simulink model "power_system"  (R2026b)
settings: Solver=VariableStepAuto  StopTime=param.sim.simlength
model workspace (MAT data in the model file):
  phi = 0.785398163397
values from neighbouring files (symbols this model uses):
  param = struct()    [init_model.m]
undefined symbols (not defined in the file or in its folder): dmavg_flt, simple_moving_average_filter
libraries: fl_lib x37, nesl_utility x22, single_phase_transformer_lib x3, saturable_single_phase_transformer x3, power_meter_iec x2, three_phase_transformer_lib x2, eeGeneralControl x2, moving_average_filter x1, moving_average_filter_cc x1, simulink x1, three_phase_voltage_with_frt_emulator x1, three_phase_rl_load x1
(part 1 of 2)
settings Model: Creator=dbagn  LastModifiedBy=d.bagnara
settings SFSimCC: SimCustomHeaderCode=|
  | #include "rpi.h"
  | #include "mavgflt.h"
  | #include "mavgflt_simulink.h"
  | #include "mavgflts.h"
  | #include "mavgflts_simulink.h"
  | #include "dsmavgflt.h"
  | #include "dsmavgflt_simulink.h"
  | #include "bemf_obsv.h"
  | #include "bemf_obsv_simulink.h"
  | #include "bemf_obsv_load_est.h"
  | #include "bemf_obsv_load_est_simulink.h"
  | #include "dqvector_pi.h"
  | #include "dqvector_pi_simulink.h"
  | #include "sv_pwm_simulink.h"
  | #include "sv_pwm.h"
  | #include "first_harmonic_tracker.h"
  | #include "first_harmonic_tracker_simulink.h"
  | #include "dqpll_thyr.h"
  | #include "dqpll_thyr_simulink.h"
  | #include "dqpll_grid.h"
  | #include "dqpll_grid_simulink.h"
  | #include "linear_double_integrator_observer_simulink.h"
  | #include "linear_double_integrator_observer.h"
settings SFSimCC: SimUserIncludeDirs=|
  | include
  | src
settings SFSimCC: SimUserSources=|
  | "rpi.c"
  | "mavgflt_simulink.c"
  | "mavgflt.c"
  | "mavgflts_simulink.c"
  | "mavgflts.c"
  | "dsmavgflt_simulink.c"
  | "dsmavgflt.c"
  | "bemf_obsv_simulink.c"
  | "bemf_obsv.c"
  | "bemf_obsv_load_est_simulink.c"
  | "bemf_obsv_load_est.c"
  | "dqvector_pi.c"
  | "dqvector_pi_simulink.c"
  | "sv_pwm_simulink.c"
  | "sv_pwm.c"
  | "first_harmonic_tracker_simulink.c"
  | "first_harmonic_tracker.c"
  | "dqpll_thyr_simulink.c"
  | "dqpll_thyr.c"
  | "dqpll_grid_simulink.c"
  | "dqpll_grid.c"
  | "linear_double_integrator_observer_simulink.c"
  | "linear_double_integrator_observer.c"
settings SimscapeCC: SimscapeUseEnergyAccounting=off

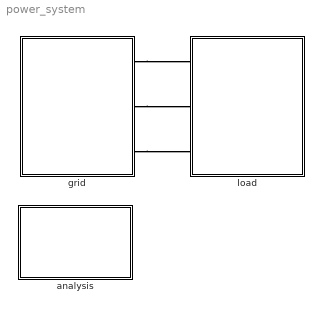
== system power_system ==
  analysis : Subsystem
  grid : Subsystem
  load : Subsystem
  connections:
  grid/RConn1 -- load/LConn1
  grid/RConn2 -- load/LConn2
  grid/RConn3 -- load/LConn3

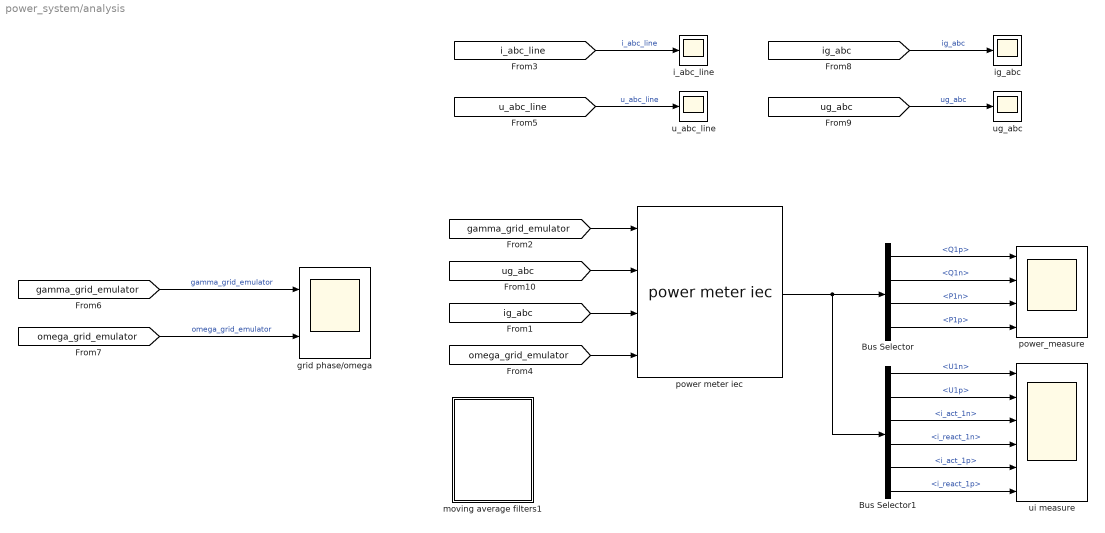
== system power_system/analysis ==
  Bus Selector : BusSelector  OutputSignals=Q1p,Q1n,P1n,P1p
  Bus Selector1 : BusSelector  OutputSignals=U1n,U1p,i_act_1n,i_react_1n,i_act_1p,i_react_1p
  grid phase/omega : Scope  NumInputPorts=2
      settings: ActiveDisplayYMinimum=-3.926953707550084  ActiveDisplayYMaximum=3.9269067422486352  DataLoggingVariableName=ScopeData3
  i_abc_line : Scope
      settings: ActiveDisplayYMinimum=-68.948090283299308  ActiveDisplayYMaximum=59.727285723031869  DataLoggingVariableName=ScopeData4
  ig_abc : Scope
      settings: ActiveDisplayYMinimum=-1  ActiveDisplayYMaximum=1  DataLoggingVariableName=ScopeData6
  moving average filters1 : Subsystem
  power meter iec : power_meter_iec/power meter iec  period=10/param.grid.emu.fgrid_nom  ts=param.glb_time.tc  enable_time=0.025
  power_measure : Scope  NumInputPorts=4
      settings: ActiveDisplayYMinimum=-20130.529238289768  ActiveDisplayYMaximum=181174.76314460795
  u_abc_line : Scope
      settings: ActiveDisplayYMinimum=-704.22830105013838  ActiveDisplayYMaximum=704.22830105010917  DataLoggingVariableName=ScopeData5
  ug_abc : Scope
      settings: ActiveDisplayYMinimum=-698.03378054285679  ActiveDisplayYMaximum=698.02521447934464  DataLoggingVariableName=ScopeData7
  ui measure : Scope  NumInputPorts=6
      settings: ActiveDisplayString=6  ActiveDisplayYMinimum=48.674141527663735  ActiveDisplayYMaximum=144.89470062623792
  wires:
  Bus Selector1/5 -> ui measure/5  "<i_act_1p>"
  Bus Selector/2 -> power_measure/2  "<Q1n>"
  [u_abc_line] -> u_abc_line/1  "u_abc_line"
  [i_abc_line] -> i_abc_line/1  "i_abc_line"
  [ig_abc] -> ig_abc/1  "ig_abc"
  [ug_abc] -> ug_abc/1  "ug_abc"
  Bus Selector1/3 -> ui measure/3  "<i_act_1n>"
  Bus Selector/1 -> power_measure/1  "<Q1p>"
  Bus Selector1/6 -> ui measure/6  "<i_react_1p>"
  Bus Selector1/4 -> ui measure/4  "<i_react_1n>"
  [ug_abc] -> power meter iec/2
  Bus Selector/3 -> power_measure/3  "<P1n>"
  [omega_grid_emulator] -> power meter iec/4
  [ig_abc] -> power meter iec/3
  [gamma_grid_emulator] -> power meter iec/1
  Bus Selector1/1 -> ui measure/1  "<U1n>"
  Bus Selector/4 -> power_measure/4  "<P1p>"
  [omega_grid_emulator] -> grid phase/omega/2  "omega_grid_emulator"
  [gamma_grid_emulator] -> grid phase/omega/1  "gamma_grid_emulator"
  power meter iec/1 -> Bus Selector/1, Bus Selector1/1
  Bus Selector1/2 -> ui measure/2  "<U1p>"

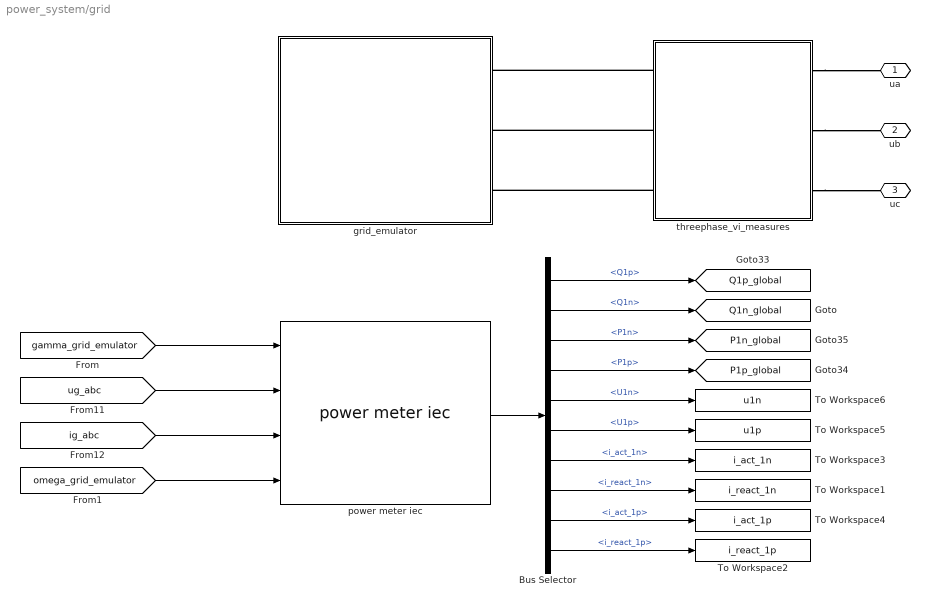
== system power_system/grid ==
  Bus Selector : BusSelector  OutputSignals=Q1p,Q1n,P1n,P1p,U1n,U1p,i_act_1n,i_react_1n,i_act_1p,i_react_1p
  To Workspace1 : ToWorkspace  VariableName=i_react_1n  SampleTime=param.glb_time.ts_afe
      settings: MaxDataPoints=param.glb_time.Ns_afe
  To Workspace2 : ToWorkspace  VariableName=i_react_1p  SampleTime=param.glb_time.ts_afe
      settings: MaxDataPoints=param.glb_time.Ns_afe
  To Workspace3 : ToWorkspace  VariableName=i_act_1n  SampleTime=param.glb_time.ts_afe
      settings: MaxDataPoints=param.glb_time.Ns_afe
  To Workspace4 : ToWorkspace  VariableName=i_act_1p  SampleTime=param.glb_time.ts_afe
      settings: MaxDataPoints=param.glb_time.Ns_afe
  To Workspace5 : ToWorkspace  VariableName=u1p  SampleTime=param.glb_time.ts_afe
      settings: MaxDataPoints=param.glb_time.Ns_afe
  To Workspace6 : ToWorkspace  VariableName=u1n  SampleTime=param.glb_time.ts_afe
      settings: MaxDataPoints=param.glb_time.Ns_afe
  grid_emulator : Subsystem
  power meter iec : power_meter_iec/power meter iec  period=pi/param.grid.emu.omega_grid_nom  ts=param.glb_time.tc  enable_time=0.025
  threephase_vi_measures : Subsystem
  ua : PMIOPort  Side=Right
  ub : PMIOPort  Port=2  Side=Right
  uc : PMIOPort  Port=3  Side=Right
  tag scope: P1n_global=global, P1p_global=global, Q1n_global=global, Q1p_global=global
  wires:
  power meter iec/1 -> Bus Selector/1
  Bus Selector/1 -> [Q1p_global]  "<Q1p>"
  Bus Selector/2 -> [Q1n_global]  "<Q1n>"
  Bus Selector/3 -> [P1n_global]  "<P1n>"
  Bus Selector/4 -> [P1p_global]  "<P1p>"
  Bus Selector/5 -> To Workspace6/1  "<U1n>"
  Bus Selector/6 -> To Workspace5/1  "<U1p>"
  Bus Selector/7 -> To Workspace3/1  "<i_act_1n>"
  Bus Selector/8 -> To Workspace1/1  "<i_react_1n>"
  Bus Selector/9 -> To Workspace4/1  "<i_act_1p>"
  Bus Selector/10 -> To Workspace2/1  "<i_react_1p>"
  [gamma_grid_emulator] -> power meter iec/1
  [ug_abc] -> power meter iec/2
  [ig_abc] -> power meter iec/3
  [omega_grid_emulator] -> power meter iec/4
  connections:
  threephase_vi_measures/LConn3 -- grid_emulator/RConn3
  threephase_vi_measures/LConn1 -- grid_emulator/RConn1
  threephase_vi_measures/RConn2 -- ub/RConn1
  threephase_vi_measures/LConn2 -- grid_emulator/RConn2
  threephase_vi_measures/RConn1 -- ua/RConn1
  threephase_vi_measures/RConn3 -- uc/RConn1

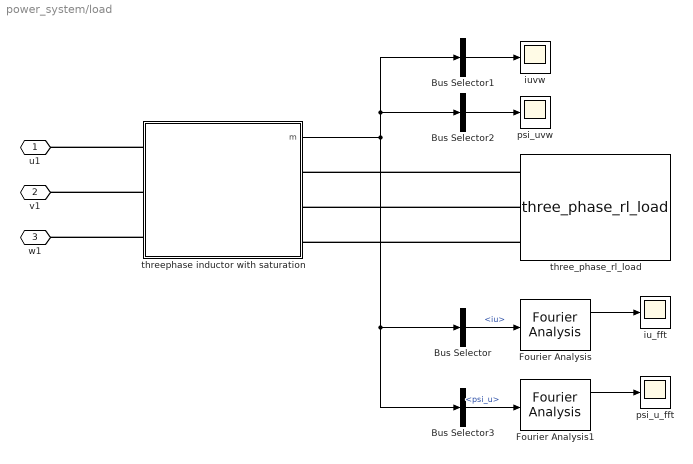
== system power_system/load ==
  Bus Selector : BusSelector  OutputSignals=iu
  Bus Selector1 : BusSelector  OutputSignals=iu,iv,iw  OutputAsBus=on
  Bus Selector2 : BusSelector  OutputSignals=psi_u,psi_v,psi_w  OutputAsBus=on
  Bus Selector3 : BusSelector  OutputSignals=psi_u
  Fourier Analysis : eeGeneralControl/Fourier Analysis  f=50  n=[3, 5, 7, 11]  M0=1  Ph0=0  BufferSize=8192  Ts=param.glb_time.ts_afe
      settings: LibrarySourceBlock=ee_sl_lib/General Control/Fourier Analysis
  Fourier Analysis1 : eeGeneralControl/Fourier Analysis  f=50  n=[3, 5, 7, 11]  M0=1  Ph0=0  BufferSize=8192  Ts=param.glb_time.ts_afe
      settings: LibrarySourceBlock=ee_sl_lib/General Control/Fourier Analysis
  iu_fft : Scope
      settings: ActiveDisplayYMinimum=-45.991562692326895  ActiveDisplayYMaximum=413.93793972331429  DataLoggingVariableName=ScopeData9
  iuvw : Scope
      settings: ActiveDisplayYMinimum=-661.72456988619081  ActiveDisplayYMaximum=615.81940216615919  DataLoggingVariableName=ScopeData8
  psi_u_fft : Scope
      settings: ActiveDisplayYMinimum=-0.2430744341634945  ActiveDisplayYMaximum=0.35456280363081638  DataLoggingVariableName=ScopeData11
  psi_uvw : Scope
      settings: ActiveDisplayYMinimum=-0.33417090779252678  ActiveDisplayYMaximum=0.310988798093905  DataLoggingVariableName=ScopeData10
  three_phase_rl_load : three_phase_rl_load/three_phase_rl_load  Ls1_load_m=param.load.Ls_load(1)  Rs1_load_m=param.load.Rs_load(1)  Ls2_load_m=param.load.Ls_load(2)  Rs2_load_m=param.load.Rs_load(2)  Ls3_load_m=param.load.Ls_load(3)  Rs3_load_m=param.load.Rs_load(3)
  threephase inductor with saturation : Subsystem  mask{LFu_m=param.load.ind.LFu, Rs_m=param.load.ind.Rs, LFu0_m=param.load.ind.LFu0, Rs0_m=param.load.ind.Rs0, isat_m=param.load.ind.isat}
      mask prompts: LFu_m "Positive Sequence Inductance [H]"; Rs_m "Positive Sequence Resistance [Ohm]"; LFu0_m "Zero Sequence Inductance [H]"; Rs0_m "Zero Sequence Resistance [Ohm]"; isat_m "Saturation Current [Arms]"
      mask Display:
      | disp('3P~ind with sat');
      | 
      | port_label('output', 1, 'm');
      | 
      | port_label('lconn', 1, 'u1');
      | port_label('lconn', 2, 'v1');
      | port_label('lconn', 3, 'w1');
      | port_label('rconn', 1, 'u2');
      | port_label('rconn', 2, 'v2');
      | port_label('rconn', 3, 'w2');
  u1 : PMIOPort  Side=Left
  v1 : PMIOPort  Port=2  Side=Left
  w1 : PMIOPort  Port=3  Side=Left
  wires:
  Bus Selector/1 -> Fourier Analysis/1  "<iu>"
  Fourier Analysis/1 -> iu_fft/1
  Bus Selector1/1 -> iuvw/1
  Bus Selector2/1 -> psi_uvw/1
  threephase inductor with saturation/1(m) -> Bus Selector2/1, Bus Selector1/1, Bus Selector3/1, Bus Selector/1
  Fourier Analysis1/1 -> psi_u_fft/1
  Bus Selector3/1 -> Fourier Analysis1/1  "<psi_u>"
  connections:
  threephase inductor with saturation/LConn1 -- u1/RConn1
  threephase inductor with saturation/LConn2 -- v1/RConn1
  threephase inductor with saturation/LConn3 -- w1/RConn1
  three_phase_rl_load/LConn1 -- threephase inductor with saturation/RConn1
  three_phase_rl_load/LConn2 -- threephase inductor with saturation/RConn2
  three_phase_rl_load/LConn3 -- threephase inductor with saturation/RConn3

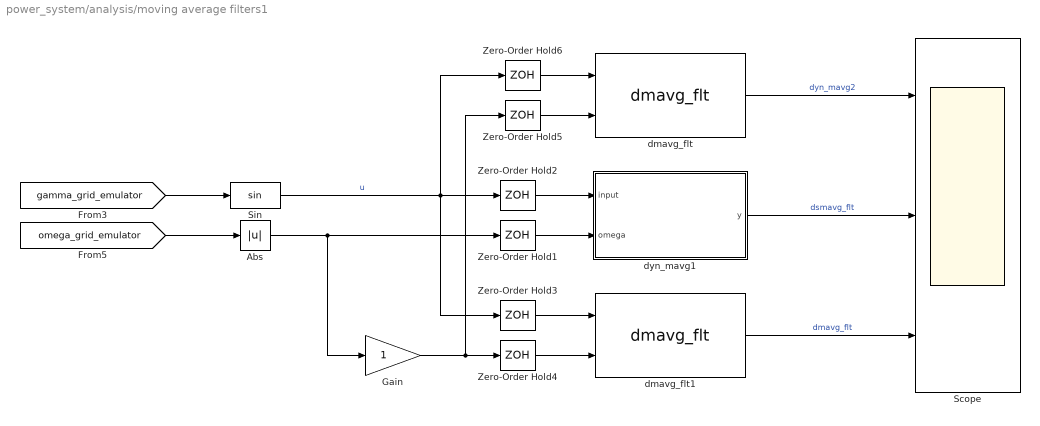
== system power_system/analysis/moving average filters1 ==
  Abs : Abs  SaturateOnIntegerOverflow=off
  Gain : Gain
  Scope : Scope  NumInputPorts=3
      settings: ActiveDisplayYMinimum=-1.2499809265136719  ActiveDisplayYMaximum=1.2499809265136719  DataLoggingVariableName=ScopeData2
  Sin : Trigonometry
  Zero-Order Hold{1..6} (6 alike) : ZeroOrderHold  SampleTime=param.glb_time.ts_afe
  dmavg_flt : moving_average_filter/dmavg_flt  ts=param.glb_time.ts_afe  enable_time=0.025
  dmavg_flt1 : moving_average_filter_cc/dmavg_flt  instance=0  ts=param.glb_time.ts_afe  enable_time=0.025
  dyn_mavg1 : Subsystem  AncestorBlock=simple_moving_average_filter/dmavg_flt  mask{ts=param.glb_time.ts_afe}
      mask prompts: ts "sampling time (s)"
      mask Display:
      | disp('dyn_mavg_flt');
      | port_label('input', 1, 'input');
      | port_label('input', 2, 'omega');
      | port_label('output', 1, 'output');
  wires:
  dyn_mavg1/1(y) -> Scope/2  "dsmavg_flt"
  Zero-Order Hold3/1 -> dmavg_flt1/1
  [gamma_grid_emulator] -> Sin/1
  Zero-Order Hold1/1 -> dyn_mavg1/2(omega)
  Zero-Order Hold4/1 -> dmavg_flt1/2
  dmavg_flt1/1 -> Scope/3  "dmavg_flt"
  [omega_grid_emulator] -> Abs/1
  Zero-Order Hold2/1 -> dyn_mavg1/1(input)
  Sin/1 -> Zero-Order Hold6/1, Zero-Order Hold3/1, Zero-Order Hold2/1  "u"
  Abs/1 -> Zero-Order Hold1/1, Gain/1
  Gain/1 -> Zero-Order Hold5/1, Zero-Order Hold4/1
  Zero-Order Hold6/1 -> dmavg_flt/1
  Zero-Order Hold5/1 -> dmavg_flt/2
  dmavg_flt/1 -> Scope/1  "dyn_mavg2"

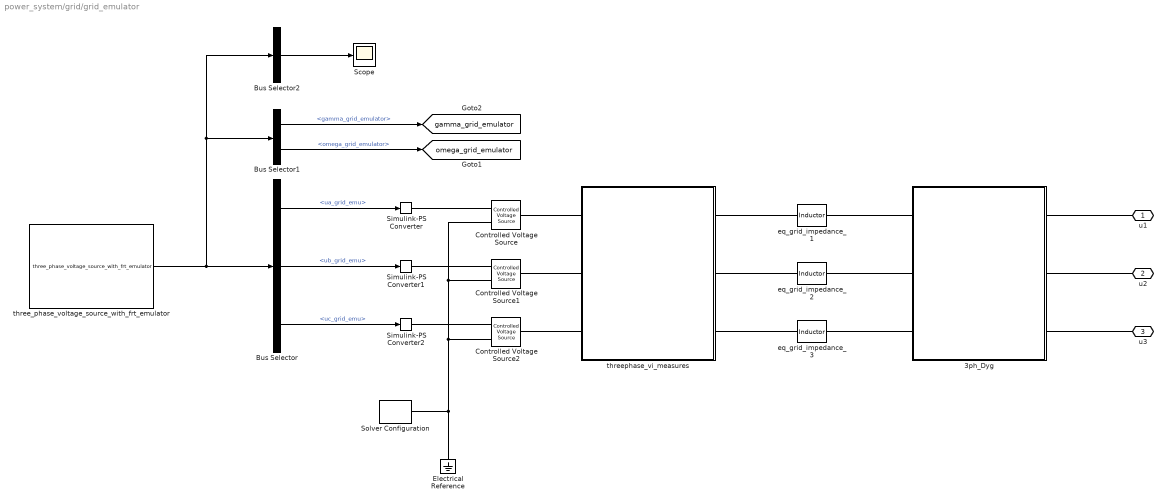
== system power_system/grid/grid_emulator ==
  3ph_Dyg : Subsystem
  Bus Selector : BusSelector  OutputSignals=ua_grid_emu,ub_grid_emu,uc_grid_emu
  Bus Selector1 : BusSelector  OutputSignals=gamma_grid_emulator,omega_grid_emulator
  Bus Selector2 : BusSelector  OutputSignals=vp_xi,vp_eta,vn_xi,vn_eta  OutputAsBus=on
  Controlled Voltage Source : fl_lib/Electrical/Electrical Sources/Controlled Voltage Source
  Controlled Voltage Source1 : fl_lib/Electrical/Electrical Sources/Controlled Voltage Source
  Controlled Voltage Source2 : fl_lib/Electrical/Electrical Sources/Controlled Voltage Source
  Electrical Reference : fl_lib/Electrical/Electrical Elements/Electrical Reference
  Scope : Scope
      settings: ActiveDisplayYMinimum=-323.94501848294675  ActiveDisplayYMaximum=661.97460298693193  DataLoggingVariableName=ScopeData12
  Simulink-PS Converter : nesl_utility/Simulink-PS Converter  PhysicalDomain=network_engine_domain  SubClassName=ps_input  LeftPortType=input  RightPortType=output  PseudoPeriodic=off  Frequencies=[]  NoiseDistribution=none  NoiseParameters=[]  Unit=V  AffineConversion=on  FilteringAndDerivatives=provide  SimscapeFilterOrder=1  InputFilterTimeConstant=0.001  UdotUserProvided=0
  Simulink-PS Converter1 : nesl_utility/Simulink-PS Converter  PhysicalDomain=network_engine_domain  SubClassName=ps_input  LeftPortType=input  RightPortType=output  PseudoPeriodic=off  Frequencies=[]  NoiseDistribution=none  NoiseParameters=[]  Unit=V  AffineConversion=on  FilteringAndDerivatives=provide  SimscapeFilterOrder=1  InputFilterTimeConstant=0.001  UdotUserProvided=0
  Simulink-PS Converter2 : nesl_utility/Simulink-PS Converter  PhysicalDomain=network_engine_domain  SubClassName=ps_input  LeftPortType=input  RightPortType=output  PseudoPeriodic=off  Frequencies=[]  NoiseDistribution=none  NoiseParameters=[]  Unit=V  AffineConversion=on  FilteringAndDerivatives=provide  SimscapeFilterOrder=1  InputFilterTimeConstant=0.001  UdotUserProvided=0
  Solver Configuration : nesl_utility/Solver Configuration  PhysicalDomain=network_engine_domain  SubClassName=solver  LeftPortType=input  RightPortType=generic  Tones=[]  Harmonics=[]  SimulateNoise=off  Profile=off  UseLocalSampling=off  EnableSwitchedLinearOptims=on  FrequencyDomain=off  UseCCode=off  RelTol=0.001  AbsTol=0.001  MinStep=1e-09  ToWorkspace=off  RevertToSquareIcSolve=off  NumHomotopyIterations=100  PhasorMode=off  PhasorModeNumHarmonics=1  ConsistencySolver=NEWTON_FTOL  CanonicalOrdering=UNORDERED  OptimizeIntermediates=UNOPTIMIZED  MulticoreSolverChoice=BACKWARD_EULER  IndexReductionMethod=DerivativeReplacement  DoDC=on  ResidualTolerance=1e-3  ConsistencyTolSource=GLOBAL  ConsistencyAbsTol=0.001  ConsistencyRelTol=0.001  ConsistencyTolFactor=0.001  UseLocalSolver=on  LocalSolverChoice=NE_BACKWARD_EULER_ADVANCER  ResolveIndetEquations=on  FunctionEvalNumThread=1  LocalSolverSampleTime=param.glb_time.tc  DoFixedCost=on  MaxNonlinIter=param.sim.nonlinear_iterations  MaxModeIter=2  ComputeImpulses=off  ImpulseIterations=2  LinearAlgebra=auto  LinearAlgebraNumThread=0  EquationFormulation=NE_TIME_EF  DelaysMemoryBudget=1024  AutomaticFiltering=on  FilteringTimeConstant=0.001  PartitionStorageMethod=AS_NEEDED  PartitionMemoryBudget=1024  PartitionMethod=BALANCED  MultibodyUseLocalSolver=off  MultibodyLocalSolverChoice=ODE1  MultibodyLocalSolverSampleTime=0.001
  eq_grid_impedance_1 : fl_lib/Electrical/Electrical Elements/Inductor  l=param.grid.emu.eq_grid_inductance H  r=param.grid.emu.eq_grid_resistance Ohm  g=1e-9 1/Ohm  i_specify=off  i_priority=None  i=0 A  i_nominal_specify=off  i_nominal_value=1  i_nominal_unit=A  v_specify=off  v_priority=None  v=0 V  v_nominal_specify=off  v_nominal_value=1  v_nominal_unit=V  i_L_specify=off  i_L_priority=High  i_L=0 A  i_L_nominal_specify=off  i_L_nominal_value=1  i_L_nominal_unit=A
  eq_grid_impedance_2 : fl_lib/Electrical/Electrical Elements/Inductor  l=param.grid.emu.eq_grid_inductance H  r=param.grid.emu.eq_grid_resistance Ohm  g=1e-9 1/Ohm  i_specify=off  i_priority=None  i=0 A  i_nominal_specify=off  i_nominal_value=1  i_nominal_unit=A  v_specify=off  v_priority=None  v=0 V  v_nominal_specify=off  v_nominal_value=1  v_nominal_unit=V  i_L_specify=off  i_L_priority=High  i_L=0 A  i_L_nominal_specify=off  i_L_nominal_value=1  i_L_nominal_unit=A
  eq_grid_impedance_3 : fl_lib/Electrical/Electrical Elements/Inductor  l=param.grid.emu.eq_grid_inductance H  r=param.grid.emu.eq_grid_resistance Ohm  g=1e-9 1/Ohm  i_specify=off  i_priority=None  i=0 A  i_nominal_specify=off  i_nominal_value=1  i_nominal_unit=A  v_specify=off  v_priority=None  v=0 V  v_nominal_specify=off  v_nominal_value=1  v_nominal_unit=V  i_L_specify=off  i_L_priority=High  i_L=0 A  i_L_nominal_specify=off  i_L_nominal_value=1  i_L_nominal_unit=A
  three_phase_voltage_source_with_frt_emulator : three_phase_voltage_with_frt_emulator/three_phase_voltage_source_with_frt_emulator  nominal_frequency_m=param.grid.emu.fgrid_nom  nominal_voltage_m=param.grid.emu.us_primary_nom  Vemu_ref_norm_m=param.grid.emu.Vemu_ref_norm  vp_xi_pu_m=param.grid.emu.up_xi_pu_ref  vp_eta_pu_m=param.grid.emu.up_eta_pu_ref  vn_xi_pu_m=param.grid.emu.un_xi_pu_ref  vn_eta_pu_m=param.grid.emu.un_eta_pu_ref  Am=param.grid.emu.sof_50Hz.ss_c.A  Bm=param.grid.emu.sof_50Hz.ss_c.B  Cm=param.grid.emu.sof_50Hz.ss_c.C  enable_frt_1_m=param.grid.frt.enable_frt_1  enable_frt_2_m=param.grid.frt.enable_frt_2  start_time_LVRT_m=param.grid.frt.start_time_LVRT  end_time_LVRT_m=param.grid.frt.end_time_LVRT  deepPOSxi_m=param.grid.frt.deepPOSxi  deepPOSeta_m=param.grid.frt.deepPOSeta  deepNEGxi_m=param.grid.frt.deepNEGxi  deepNEGeta_m=param.grid.frt.deepNEGeta  Amplitude_U_m=param.grid.frt.Amplitude_U  Amplitude_V_m=param.grid.frt.Amplitude_V  Amplitude_W_m=param.grid.frt.Amplitude_W  t_ramp_m=param.grid.frt.t_ramp  Phase_shift_m=param.grid.frt.Phase_shift
  threephase_vi_measures : Subsystem
  u1 : PMIOPort  Side=Right
  u2 : PMIOPort  Port=2  Side=Right
  u3 : PMIOPort  Port=3  Side=Right
  tag scope: gamma_grid_emulator=global, omega_grid_emulator=global
  wires:
  Bus Selector1/2 -> [omega_grid_emulator]  "<omega_grid_emulator>"
  Bus Selector1/1 -> [gamma_grid_emulator]  "<gamma_grid_emulator>"
  Bus Selector/2 -> Simulink-PS Converter1/1  "<ub_grid_emu>"
  Bus Selector/3 -> Simulink-PS Converter2/1  "<uc_grid_emu>"
  three_phase_voltage_source_with_frt_emulator/1 -> Bus Selector1/1, Bus Selector2/1, Bus Selector/1
  Bus Selector/1 -> Simulink-PS Converter/1  "<ua_grid_emu>"
  Bus Selector2/1 -> Scope/1
  connections:
  Simulink-PS Converter/RConn1 -- Controlled Voltage Source/RConn1
  Simulink-PS Converter1/RConn1 -- Controlled Voltage Source1/RConn1
  Simulink-PS Converter2/RConn1 -- Controlled Voltage Source2/RConn1
  Controlled Voltage Source/RConn2 -- Controlled Voltage Source1/RConn2 -- Controlled Voltage Source2/RConn2 -- Electrical Reference/LConn1 -- Solver Configuration/RConn1
  3ph_Dyg/RConn1 -- u1/RConn1
  3ph_Dyg/RConn2 -- u2/RConn1
  3ph_Dyg/RConn3 -- u3/RConn1
  eq_grid_impedance_1/LConn1 -- threephase_vi_measures/RConn1
  eq_grid_impedance_2/LConn1 -- threephase_vi_measures/RConn2
  eq_grid_impedance_3/LConn1 -- threephase_vi_measures/RConn3
  Controlled Voltage Source/LConn1 -- threephase_vi_measures/LConn1
  Controlled Voltage Source1/LConn1 -- threephase_vi_measures/LConn2
  Controlled Voltage Source2/LConn1 -- threephase_vi_measures/LConn3
  3ph_Dyg/LConn1 -- eq_grid_impedance_1/RConn1
  3ph_Dyg/LConn2 -- eq_grid_impedance_2/RConn1
  3ph_Dyg/LConn3 -- eq_grid_impedance_3/RConn1

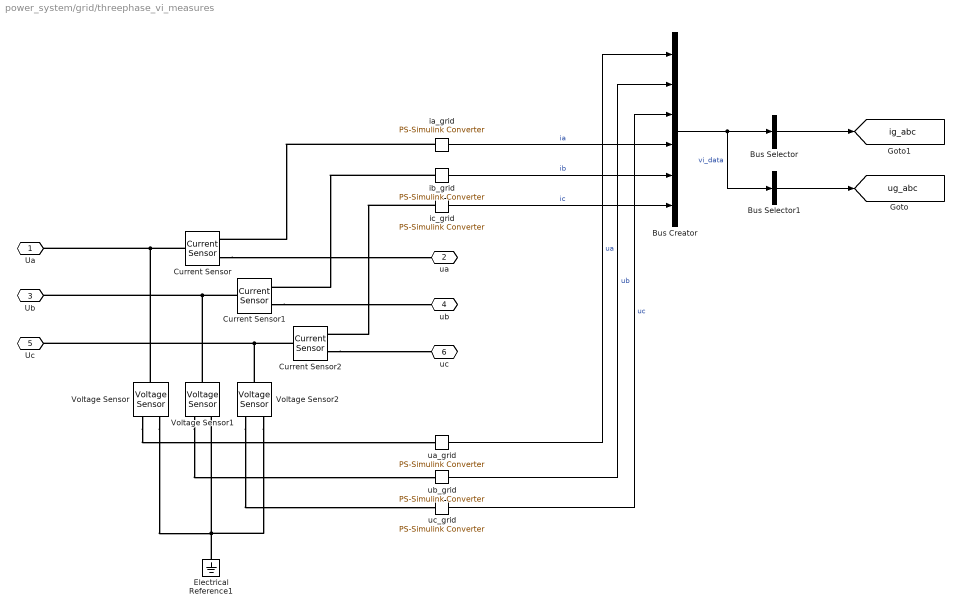
== system power_system/grid/threephase_vi_measures ==
  Bus Creator : BusCreator  Inputs=6
  Bus Selector : BusSelector  OutputSignals=ia,ib,ic  OutputAsBus=on
  Bus Selector1 : BusSelector  OutputSignals=ua,ub,uc  OutputAsBus=on
  Current Sensor : fl_lib/Electrical/Electrical Sensors/Current Sensor
  Current Sensor1 : fl_lib/Electrical/Electrical Sensors/Current Sensor
  Current Sensor2 : fl_lib/Electrical/Electrical Sensors/Current Sensor
  Electrical Reference1 : fl_lib/Electrical/Electrical Elements/Electrical Reference
  Voltage Sensor : fl_lib/Electrical/Electrical Sensors/Voltage Sensor
  Voltage Sensor1 : fl_lib/Electrical/Electrical Sensors/Voltage Sensor
  Voltage Sensor2 : fl_lib/Electrical/Electrical Sensors/Voltage Sensor
  ia_grid : nesl_utility/PS-Simulink Converter  PhysicalDomain=network_engine_domain  SubClassName=ps_output  LeftPortType=input  RightPortType=output  PseudoPeriodic=off  Frequencies=[]  VectorFormat=1-D array  Unit=A  AffineConversion=off
  ib_grid : nesl_utility/PS-Simulink Converter  PhysicalDomain=network_engine_domain  SubClassName=ps_output  LeftPortType=input  RightPortType=output  PseudoPeriodic=off  Frequencies=[]  VectorFormat=1-D array  Unit=A  AffineConversion=off
  ic_grid : nesl_utility/PS-Simulink Converter  PhysicalDomain=network_engine_domain  SubClassName=ps_output  LeftPortType=input  RightPortType=output  PseudoPeriodic=off  Frequencies=[]  VectorFormat=1-D array  Unit=A  AffineConversion=off
  ua_grid : nesl_utility/PS-Simulink Converter  PhysicalDomain=network_engine_domain  SubClassName=ps_output  LeftPortType=input  RightPortType=output  PseudoPeriodic=off  Frequencies=[]  VectorFormat=1-D array  Unit=V  AffineConversion=off
  ub_grid : nesl_utility/PS-Simulink Converter  PhysicalDomain=network_engine_domain  SubClassName=ps_output  LeftPortType=input  RightPortType=output  PseudoPeriodic=off  Frequencies=[]  VectorFormat=1-D array  Unit=V  AffineConversion=off
  uc_grid : nesl_utility/PS-Simulink Converter  PhysicalDomain=network_engine_domain  SubClassName=ps_output  LeftPortType=input  RightPortType=output  PseudoPeriodic=off  Frequencies=[]  VectorFormat=1-D array  Unit=V  AffineConversion=off
  Ua : PMIOPort  Side=Left
  ua : PMIOPort  Port=2  Side=Right
  Ub : PMIOPort  Port=3  Side=Left
  ub : PMIOPort  Port=4  Side=Right
  Uc : PMIOPort  Port=5  Side=Left
  uc : PMIOPort  Port=6  Side=Right
  tag scope: ig_abc=global, ug_abc=global
  wires:
  Bus Creator/1 -> Bus Selector1/1, Bus Selector/1  "vi_data"
  Bus Selector1/1 -> [ug_abc]
  ib_grid/1 -> Bus Creator/5  "ib"
  ia_grid/1 -> Bus Creator/4  "ia"
  ic_grid/1 -> Bus Creator/6  "ic"
  ua_grid/1 -> Bus Creator/1  "ua"
  ub_grid/1 -> Bus Creator/2  "ub"
  uc_grid/1 -> Bus Creator/3  "uc"
  Bus Selector/1 -> [ig_abc]
  connections:
  Current Sensor1/LConn1 -- Ub/RConn1 -- Voltage Sensor1/LConn1
  Electrical Reference1/LConn1 -- Voltage Sensor/RConn2 -- Voltage Sensor2/RConn2 -- Voltage Sensor1/RConn2
  Voltage Sensor/RConn1 -- ua_grid/LConn1
  Current Sensor/RConn2 -- ua/RConn1
  Voltage Sensor1/RConn1 -- ub_grid/LConn1
  Voltage Sensor2/LConn1 -- Current Sensor2/LConn1 -- Uc/RConn1
  Current Sensor/LConn1 -- Ua/RConn1 -- Voltage Sensor/LConn1
  Current Sensor1/RConn2 -- ub/RConn1
  Voltage Sensor2/RConn1 -- uc_grid/LConn1
  ib_grid/LConn1 -- Current Sensor1/RConn1
  ia_grid/LConn1 -- Current Sensor/RConn1
  ic_grid/LConn1 -- Current Sensor2/RConn1
  Current Sensor2/RConn2 -- uc/RConn1

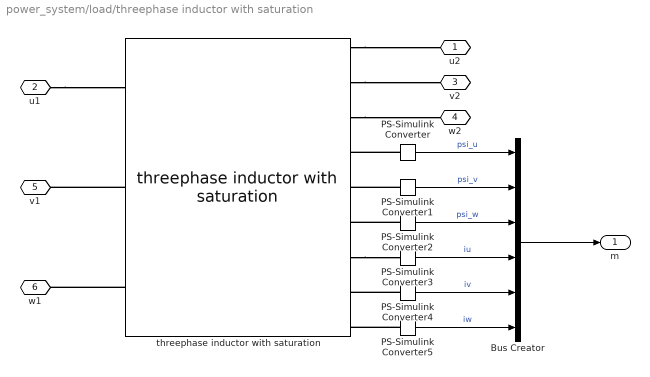
== system power_system/load/threephase inductor with saturation ==
  Bus Creator : BusCreator  Inputs=6
  PS-Simulink Converter : nesl_utility/PS-Simulink Converter  PhysicalDomain=network_engine_domain  SubClassName=ps_output  LeftPortType=input  RightPortType=output  PseudoPeriodic=off  Frequencies=[]  VectorFormat=1-D array  Unit=V*s  AffineConversion=off
  PS-Simulink Converter1 : nesl_utility/PS-Simulink Converter  PhysicalDomain=network_engine_domain  SubClassName=ps_output  LeftPortType=input  RightPortType=output  PseudoPeriodic=off  Frequencies=[]  VectorFormat=1-D array  Unit=V*s  AffineConversion=off
  PS-Simulink Converter2 : nesl_utility/PS-Simulink Converter  PhysicalDomain=network_engine_domain  SubClassName=ps_output  LeftPortType=input  RightPortType=output  PseudoPeriodic=off  Frequencies=[]  VectorFormat=1-D array  Unit=V*s  AffineConversion=off
  PS-Simulink Converter3 : nesl_utility/PS-Simulink Converter  PhysicalDomain=network_engine_domain  SubClassName=ps_output  LeftPortType=input  RightPortType=output  PseudoPeriodic=off  Frequencies=[]  VectorFormat=1-D array  Unit=A  AffineConversion=off
  PS-Simulink Converter4 : nesl_utility/PS-Simulink Converter  PhysicalDomain=network_engine_domain  SubClassName=ps_output  LeftPortType=input  RightPortType=output  PseudoPeriodic=off  Frequencies=[]  VectorFormat=1-D array  Unit=A  AffineConversion=off
  PS-Simulink Converter5 : nesl_utility/PS-Simulink Converter  PhysicalDomain=network_engine_domain  SubClassName=ps_output  LeftPortType=input  RightPortType=output  PseudoPeriodic=off  Frequencies=[]  VectorFormat=1-D array  Unit=A  AffineConversion=off
  threephase inductor with saturation : threephase_inductor_with_saturation_lib/threephase inductor with saturation  Lp=LFu_m H  L0=LFu0_m H  Rp=Rs_m Ohm  R0=Rs0_m Ohm  Lls=5e-6 H  i_base=isat_m A  uu_1_specify=off  uu_1_priority=None  uu_1=0 V  uu_1_nominal_specify=off  uu_1_nominal_value=1  uu_1_nominal_unit=V  uv_1_specify=off  uv_1_priority=None  uv_1=0 V  uv_1_nominal_specify=off  uv_1_nominal_value=1  uv_1_nominal_unit=V  uw_1_specify=off  uw_1_priority=None  uw_1=0 V  uw_1_nominal_specify=off  uw_1_nominal_value=1  uw_1_nominal_unit=V  uu_2_specify=off  uu_2_priority=None  uu_2=0 V  uu_2_nominal_specify=off  uu_2_nominal_value=1  uu_2_nominal_unit=V  uv_2_specify=off  uv_2_priority=None  uv_2=0 V  uv_2_nominal_specify=off  uv_2_nominal_value=1  uv_2_nominal_unit=V  uw_2_specify=off  uw_2_priority=None  uw_2=0 V  uw_2_nominal_specify=off  uw_2_nominal_value=1  uw_2_nominal_unit=V  iu_specify=off  iu_priority=None  iu=0 A  iu_nominal_specify=off  iu_nominal_value=1  iu_nominal_unit=A  iv_specify=off  iv_priority=None  iv=0 A  iv_nominal_specify=off  iv_nominal_value=1  iv_nominal_unit=A  iw_specify=off  iw_priority=None  iw=0 A  iw_nominal_specify=off  iw_nominal_value=1  iw_nominal_unit=A  psi_u_specify=off  psi_u_priority=High  psi_u=0 V*s  psi_u_nominal_specify=off  psi_u_nominal_value=1  psi_u_nominal_unit=V*s  psi_v_specify=off  psi_v_priority=High  psi_v=0 V*s  psi_v_nominal_specify=off  psi_v_nominal_value=1  psi_v_nominal_unit=V*s  psi_w_specify=off  psi_w_priority=Low  psi_w=0 V*s  psi_w_nominal_specify=off  psi_w_nominal_value=1  psi_w_nominal_unit=V*s  ku_La_saturation_specify=off  ku_La_saturation_priority=High  ku_La_saturation=1  ku_La_saturation_nominal_specify=off  ku_La_saturation_nominal_value=1  ku_La_saturation_nominal_unit=1  kv_La_saturation_specify=off  kv_La_saturation_priority=High  kv_La_saturation=1  kv_La_saturation_nominal_specify=off  kv_La_saturation_nominal_value=1  kv_La_saturation_nominal_unit=1  kw_La_saturation_specify=off  kw_La_saturation_priority=High  kw_La_saturation=1  kw_La_saturation_nominal_specify=off  kw_La_saturation_nominal_value=1  kw_La_saturation_nominal_unit=1  ku_Lm_saturation_specify=off  ku_Lm_saturation_priority=High  ku_Lm_saturation=1  ku_Lm_saturation_nominal_specify=off  ku_Lm_saturation_nominal_value=1  ku_Lm_saturation_nominal_unit=1  kv_Lm_saturation_specify=off  kv_Lm_saturation_priority=High  kv_Lm_saturation=1  kv_Lm_saturation_nominal_specify=off  kv_Lm_saturation_nominal_value=1  kv_Lm_saturation_nominal_unit=1  kw_Lm_saturation_specify=off  kw_Lm_saturation_priority=High  kw_Lm_saturation=1  kw_Lm_saturation_nominal_specify=off  kw_Lm_saturation_nominal_value=1  kw_Lm_saturation_nominal_unit=1  Lau_actual_specify=off  Lau_actual_priority=None  Lau_actual=0 H  Lau_actual_nominal_specify=off  Lau_actual_nominal_value=1  Lau_actual_nominal_unit=H  Lav_actual_specify=off  Lav_actual_priority=None  Lav_actual=0 H  Lav_actual_nominal_specify=off  Lav_actual_nominal_value=1  Lav_actual_nominal_unit=H  Law_actual_specify=off  Law_actual_priority=None  Law_actual=0 H  Law_actual_nominal_specify=off  Law_actual_nominal_value=1  Law_actual_nominal_unit=H  Lmu_actual_specify=off  Lmu_actual_priority=None  Lmu_actual=0 H  Lmu_actual_nominal_specify=off  Lmu_actual_nominal_value=1  Lmu_actual_nominal_unit=H  Lmv_actual_specify=off  Lmv_actual_priority=None  Lmv_actual=0 H  Lmv_actual_nominal_specify=off  Lmv_actual_nominal_value=1  Lmv_actual_nominal_unit=H  Lmw_actual_specify=off  Lmw_actual_priority=None  Lmw_actual=0 H  Lmw_actual_nominal_specify=off  Lmw_actual_nominal_value=1  Lmw_actual_nominal_unit=H  iu_pos_norm_specify=off  iu_pos_norm_priority=None  iu_pos_norm=0  iu_pos_norm_nominal_specify=off  iu_pos_norm_nominal_value=1  iu_pos_norm_nominal_unit=1  iv_pos_norm_specify=off  iv_pos_norm_priority=None  iv_pos_norm=0  iv_pos_norm_nominal_specify=off  iv_pos_norm_nominal_value=1  iv_pos_norm_nominal_unit=1  iw_pos_norm_specify=off  iw_pos_norm_priority=None  iw_pos_norm=0  iw_pos_norm_nominal_specify=off  iw_pos_norm_nominal_value=1  iw_pos_norm_nominal_unit=1
  u2 : PMIOPort  Side=Right
  u1 : PMIOPort  Port=2  Side=Left
  v2 : PMIOPort  Port=3  Side=Right
  w2 : PMIOPort  Port=4  Side=Right
  v1 : PMIOPort  Port=5  Side=Left
  w1 : PMIOPort  Port=6  Side=Left
  m : Outport
  wires:
  PS-Simulink Converter5/1 -> Bus Creator/6  "iw"
  PS-Simulink Converter4/1 -> Bus Creator/5  "iv"
  PS-Simulink Converter3/1 -> Bus Creator/4  "iu"
  PS-Simulink Converter2/1 -> Bus Creator/3  "psi_w"
  PS-Simulink Converter1/1 -> Bus Creator/2  "psi_v"
  PS-Simulink Converter/1 -> Bus Creator/1  "psi_u"
  Bus Creator/1 -> m/1
  connections:
  threephase inductor with saturation/LConn2 -- v1/RConn1
  u1/RConn1 -- threephase inductor with saturation/LConn1
  threephase inductor with saturation/LConn3 -- w1/RConn1
  threephase inductor with saturation/RConn2 -- v2/RConn1
  threephase inductor with saturation/RConn3 -- w2/RConn1
  threephase inductor with saturation/RConn1 -- u2/RConn1
  PS-Simulink Converter/LConn1 -- threephase inductor with saturation/RConn4
  PS-Simulink Converter1/LConn1 -- threephase inductor with saturation/RConn5
  PS-Simulink Converter2/LConn1 -- threephase inductor with saturation/RConn6
  threephase inductor with saturation/RConn7 -- PS-Simulink Converter3/LConn1
  PS-Simulink Converter4/LConn1 -- threephase inductor with saturation/RConn8
  PS-Simulink Converter5/LConn1 -- threephase inductor with saturation/RConn9

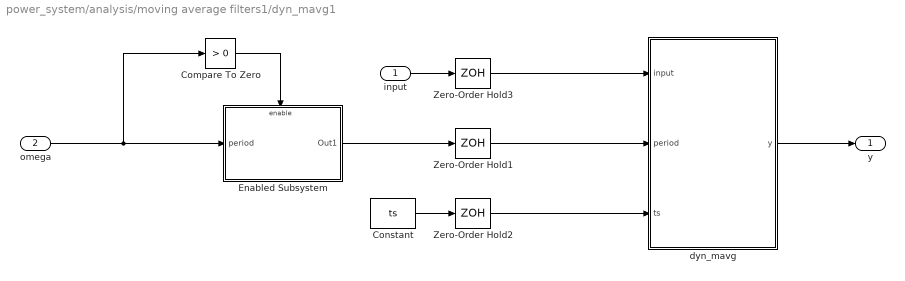
== system power_system/analysis/moving average filters1/dyn_mavg1 ==
  input : Inport
  omega : Inport  Port=2
  Compare To Zero : simulink/Logic and Bit Operations/Compare To Zero  relop=>  OutDataTypeStr=boolean
  Constant : Constant  Value=ts
  Enabled Subsystem : Subsystem  TreatAsAtomicUnit=on
  Zero-Order Hold1 : ZeroOrderHold  SampleTime=-1
  Zero-Order Hold2 : ZeroOrderHold  SampleTime=-1
  Zero-Order Hold3 : ZeroOrderHold  SampleTime=-1
  dyn_mavg : MATLAB Function  TreatAsAtomicUnit=on
  y : Outport
  wires:
  omega/1 -> Compare To Zero/1, Enabled Subsystem/1(period)
  Enabled Subsystem/1(Out1) -> Zero-Order Hold1/1
  Compare To Zero/1 -> Enabled Subsystem/Enable
  input/1 -> Zero-Order Hold3/1
  Constant/1 -> Zero-Order Hold2/1
  dyn_mavg/1(y) -> y/1
  Zero-Order Hold1/1 -> dyn_mavg/2(period)
  Zero-Order Hold3/1 -> dyn_mavg/1(input)
  Zero-Order Hold2/1 -> dyn_mavg/3(ts)

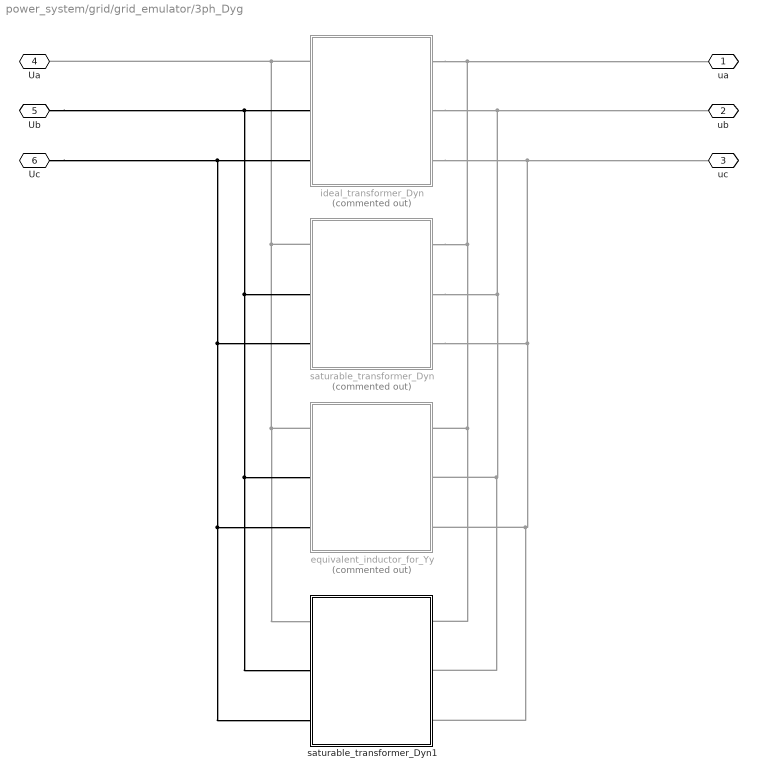
== system power_system/grid/grid_emulator/3ph_Dyg ==
  equivalent_inductor_for_Yy : Subsystem  Commented=on
  ideal_transformer_Dyn : Subsystem  Commented=on
  saturable_transformer_Dyn : Subsystem  Commented=on
  saturable_transformer_Dyn1 : Subsystem
  ua : PMIOPort  Side=Right
  ub : PMIOPort  Port=2  Side=Right
  uc : PMIOPort  Port=3  Side=Right
  Ua : PMIOPort  Port=4  Side=Left
  Ub : PMIOPort  Port=5  Side=Left
  Uc : PMIOPort  Port=6  Side=Left
  connections:
  ideal_transformer_Dyn/RConn1 -- saturable_transformer_Dyn/RConn1 -- saturable_transformer_Dyn1/RConn1 -- equivalent_inductor_for_Yy/RConn1 -- ua/RConn1
  ideal_transformer_Dyn/RConn2 -- saturable_transformer_Dyn/RConn2 -- saturable_transformer_Dyn1/RConn2 -- equivalent_inductor_for_Yy/RConn2 -- ub/RConn1
  ideal_transformer_Dyn/RConn3 -- saturable_transformer_Dyn/RConn3 -- saturable_transformer_Dyn1/RConn3 -- equivalent_inductor_for_Yy/RConn3 -- uc/RConn1
  ideal_transformer_Dyn/LConn1 -- saturable_transformer_Dyn1/LConn1 -- equivalent_inductor_for_Yy/LConn1 -- saturable_transformer_Dyn/LConn1 -- Ua/RConn1
  Ub/RConn1 -- ideal_transformer_Dyn/LConn2 -- saturable_transformer_Dyn1/LConn2 -- equivalent_inductor_for_Yy/LConn2 -- saturable_transformer_Dyn/LConn2
  Uc/RConn1 -- ideal_transformer_Dyn/LConn3 -- saturable_transformer_Dyn1/LConn3 -- equivalent_inductor_for_Yy/LConn3 -- saturable_transformer_Dyn/LConn3

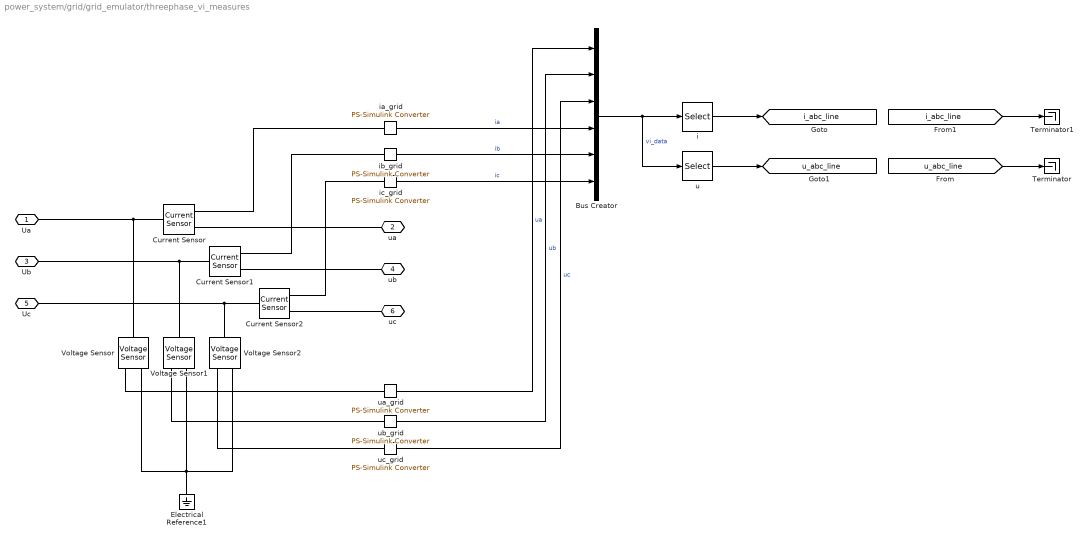
== system power_system/grid/grid_emulator/threephase_vi_measures ==
  Bus Creator : BusCreator  Inputs=6
  Current Sensor : fl_lib/Electrical/Electrical Sensors/Current Sensor
  Current Sensor1 : fl_lib/Electrical/Electrical Sensors/Current Sensor
  Current Sensor2 : fl_lib/Electrical/Electrical Sensors/Current Sensor
  Electrical Reference1 : fl_lib/Electrical/Electrical Elements/Electrical Reference
  Terminator : Terminator
  Terminator1 : Terminator
  Voltage Sensor : fl_lib/Electrical/Electrical Sensors/Voltage Sensor
  Voltage Sensor1 : fl_lib/Electrical/Electrical Sensors/Voltage Sensor
  Voltage Sensor2 : fl_lib/Electrical/Electrical Sensors/Voltage Sensor
  i : Selector  InputPortWidth=6  IndexOptions=Index vector (dialog)  Indices=[4 5 6]  OutputSizes=1  RuntimeRangeChecks=off
  ia_grid : nesl_utility/PS-Simulink Converter  PhysicalDomain=network_engine_domain  SubClassName=ps_output  LeftPortType=input  RightPortType=output  PseudoPeriodic=off  Frequencies=[]  VectorFormat=1-D array  Unit=A  AffineConversion=off
  ib_grid : nesl_utility/PS-Simulink Converter  PhysicalDomain=network_engine_domain  SubClassName=ps_output  LeftPortType=input  RightPortType=output  PseudoPeriodic=off  Frequencies=[]  VectorFormat=1-D array  Unit=A  AffineConversion=off
  ic_grid : nesl_utility/PS-Simulink Converter  PhysicalDomain=network_engine_domain  SubClassName=ps_output  LeftPortType=input  RightPortType=output  PseudoPeriodic=off  Frequencies=[]  VectorFormat=1-D array  Unit=A  AffineConversion=off
  u : Selector  InputPortWidth=6  IndexOptions=Index vector (dialog)  Indices=[1 2 3]  OutputSizes=1  RuntimeRangeChecks=off
  ua_grid : nesl_utility/PS-Simulink Converter  PhysicalDomain=network_engine_domain  SubClassName=ps_output  LeftPortType=input  RightPortType=output  PseudoPeriodic=off  Frequencies=[]  VectorFormat=1-D array  Unit=V  AffineConversion=off
  ub_grid : nesl_utility/PS-Simulink Converter  PhysicalDomain=network_engine_domain  SubClassName=ps_output  LeftPortType=input  RightPortType=output  PseudoPeriodic=off  Frequencies=[]  VectorFormat=1-D array  Unit=V  AffineConversion=off
  uc_grid : nesl_utility/PS-Simulink Converter  PhysicalDomain=network_engine_domain  SubClassName=ps_output  LeftPortType=input  RightPortType=output  PseudoPeriodic=off  Frequencies=[]  VectorFormat=1-D array  Unit=V  AffineConversion=off
  Ua : PMIOPort  Side=Left
  ua : PMIOPort  Port=2  Side=Right
  Ub : PMIOPort  Port=3  Side=Left
  ub : PMIOPort  Port=4  Side=Right
  Uc : PMIOPort  Port=5  Side=Left
  uc : PMIOPort  Port=6  Side=Right
  tag scope: i_abc_line=global, u_abc_line=global
  wires:
  Bus Creator/1 -> i/1, u/1  "vi_data"
  ib_grid/1 -> Bus Creator/5  "ib"
  ia_grid/1 -> Bus Creator/4  "ia"
  ic_grid/1 -> Bus Creator/6  "ic"
  ua_grid/1 -> Bus Creator/1  "ua"
  ub_grid/1 -> Bus Creator/2  "ub"
  uc_grid/1 -> Bus Creator/3  "uc"
  i/1 -> [i_abc_line]
  u/1 -> [u_abc_line]
  [u_abc_line] -> Terminator/1
  [i_abc_line] -> Terminator1/1
  connections:
  Current Sensor1/LConn1 -- Ub/RConn1 -- Voltage Sensor1/LConn1
  Electrical Reference1/LConn1 -- Voltage Sensor/RConn2 -- Voltage Sensor2/RConn2 -- Voltage Sensor1/RConn2
  Voltage Sensor/RConn1 -- ua_grid/LConn1
  Current Sensor/RConn2 -- ua/RConn1
  Voltage Sensor1/RConn1 -- ub_grid/LConn1
  Voltage Sensor2/LConn1 -- Current Sensor2/LConn1 -- Uc/RConn1
  Current Sensor/LConn1 -- Ua/RConn1 -- Voltage Sensor/LConn1
  Current Sensor1/RConn2 -- ub/RConn1
  Voltage Sensor2/RConn1 -- uc_grid/LConn1
  ib_grid/LConn1 -- Current Sensor1/RConn1
  ia_grid/LConn1 -- Current Sensor/RConn1
  ic_grid/LConn1 -- Current Sensor2/RConn1
  Current Sensor2/RConn2 -- uc/RConn1

== system power_system/analysis/moving average filters1/dyn_mavg1/Enabled Subsystem ==
  period : Inport
  Enable : EnablePort
  Constant2 : Constant
  Divide : Product  Inputs=*/
  Gain1 : Gain  Gain=1/(2*pi)
  Out1 : Outport
  wires:
  Divide/1 -> Out1/1  "period"
  Gain1/1 -> Divide/2
  period/1 -> Gain1/1  "omega"
  Constant2/1 -> Divide/1

== system power_system/grid/grid_emulator/3ph_Dyg/equivalent_inductor_for_Yy ==
  Inductor : fl_lib/Electrical/Electrical Elements/Inductor  l=2*param.grid.emu.trafo.Ld2 H  r=2*param.grid.emu.trafo.Rd2 Ohm  g=1e-9 1/Ohm  i_specify=off  i_priority=None  i=0 A  i_nominal_specify=off  i_nominal_value=1  i_nominal_unit=A  v_specify=off  v_priority=None  v=0 V  v_nominal_specify=off  v_nominal_value=1  v_nominal_unit=V  i_L_specify=off  i_L_priority=High  i_L=0 A  i_L_nominal_specify=off  i_L_nominal_value=1  i_L_nominal_unit=A
  Inductor1 : fl_lib/Electrical/Electrical Elements/Inductor  l=2*param.grid.emu.trafo.Ld2 H  r=2*param.grid.emu.trafo.Rd2 Ohm  g=1e-9 1/Ohm  i_specify=off  i_priority=None  i=0 A  i_nominal_specify=off  i_nominal_value=1  i_nominal_unit=A  v_specify=off  v_priority=None  v=0 V  v_nominal_specify=off  v_nominal_value=1  v_nominal_unit=V  i_L_specify=off  i_L_priority=High  i_L=0 A  i_L_nominal_specify=off  i_L_nominal_value=1  i_L_nominal_unit=A
  Inductor2 : fl_lib/Electrical/Electrical Elements/Inductor  l=2*param.grid.emu.trafo.Ld2 H  r=2*param.grid.emu.trafo.Rd2 Ohm  g=1e-9 1/Ohm  i_specify=off  i_priority=None  i=0 A  i_nominal_specify=off  i_nominal_value=1  i_nominal_unit=A  v_specify=off  v_priority=None  v=0 V  v_nominal_specify=off  v_nominal_value=1  v_nominal_unit=V  i_L_specify=off  i_L_priority=High  i_L=0 A  i_L_nominal_specify=off  i_L_nominal_value=1  i_L_nominal_unit=A
  ua : PMIOPort  Side=Right
  ub : PMIOPort  Port=2  Side=Right
  uc : PMIOPort  Port=3  Side=Right
  Ua : PMIOPort  Port=4  Side=Left
  Ub : PMIOPort  Port=5  Side=Left
  Uc : PMIOPort  Port=6  Side=Left
  connections:
  Inductor/RConn1 -- ua/RConn1
  Inductor/LConn1 -- Ua/RConn1
  Inductor2/LConn1 -- Uc/RConn1
  Inductor1/LConn1 -- Ub/RConn1
  ub/RConn1 -- Inductor1/RConn1
  uc/RConn1 -- Inductor2/RConn1

== system power_system/grid/grid_emulator/3ph_Dyg/ideal_transformer_Dyn ==
  Electrical Reference1 : fl_lib/Electrical/Electrical Elements/Electrical Reference
  ph1 : single_phase_transformer_lib/single phase transformer  Lm=param.grid.emu.trafo.Lm1 H  n1=param.grid.emu.trafo.n1  n2=param.grid.emu.trafo.n2  Rd1=param.grid.emu.trafo.Rd1 Ohm  Rd2=param.grid.emu.trafo.Rd2 Ohm  Ld1=param.grid.emu.trafo.Ld1 H  Ld2=param.grid.emu.trafo.Ld2 H  Rfe=param.grid.emu.trafo.Rfe1 Ohm  phi_specify=off  phi_priority=None  phi=0 V*s  phi_nominal_specify=off  phi_nominal_value=1  phi_nominal_unit=V*s  i1_specify=off  i1_priority=None  i1=0 A  i1_nominal_specify=off  i1_nominal_value=1  i1_nominal_unit=A  i2_specify=off  i2_priority=None  i2=0 A  i2_nominal_specify=off  i2_nominal_value=1  i2_nominal_unit=A  ife_specify=off  ife_priority=None  ife=0 A  ife_nominal_specify=off  ife_nominal_value=1  ife_nominal_unit=A  u1_specify=off  u1_priority=None  u1=0 V  u1_nominal_specify=off  u1_nominal_value=1  u1_nominal_unit=V  u2_specify=off  u2_priority=None  u2=0 V  u2_nominal_specify=off  u2_nominal_value=1  u2_nominal_unit=V
  ph2 : single_phase_transformer_lib/single phase transformer  Lm=param.grid.emu.trafo.Lm1 H  n1=param.grid.emu.trafo.n1  n2=param.grid.emu.trafo.n2  Rd1=param.grid.emu.trafo.Rd1 Ohm  Rd2=param.grid.emu.trafo.Rd2 Ohm  Ld1=param.grid.emu.trafo.Ld1 H  Ld2=param.grid.emu.trafo.Ld2 H  Rfe=param.grid.emu.trafo.Rfe1 Ohm  phi_specify=off  phi_priority=None  phi=0 V*s  phi_nominal_specify=off  phi_nominal_value=1  phi_nominal_unit=V*s  i1_specify=off  i1_priority=None  i1=0 A  i1_nominal_specify=off  i1_nominal_value=1  i1_nominal_unit=A  i2_specify=off  i2_priority=None  i2=0 A  i2_nominal_specify=off  i2_nominal_value=1  i2_nominal_unit=A  ife_specify=off  ife_priority=None  ife=0 A  ife_nominal_specify=off  ife_nominal_value=1  ife_nominal_unit=A  u1_specify=off  u1_priority=None  u1=0 V  u1_nominal_specify=off  u1_nominal_value=1  u1_nominal_unit=V  u2_specify=off  u2_priority=None  u2=0 V  u2_nominal_specify=off  u2_nominal_value=1  u2_nominal_unit=V
  ph3 : single_phase_transformer_lib/single phase transformer  Lm=param.grid.emu.trafo.Lm1 H  n1=param.grid.emu.trafo.n1  n2=param.grid.emu.trafo.n2  Rd1=param.grid.emu.trafo.Rd1 Ohm  Rd2=param.grid.emu.trafo.Rd2 Ohm  Ld1=param.grid.emu.trafo.Ld1 H  Ld2=param.grid.emu.trafo.Ld2 H  Rfe=param.grid.emu.trafo.Rfe1 Ohm  phi_specify=off  phi_priority=None  phi=0 V*s  phi_nominal_specify=off  phi_nominal_value=1  phi_nominal_unit=V*s  i1_specify=off  i1_priority=None  i1=0 A  i1_nominal_specify=off  i1_nominal_value=1  i1_nominal_unit=A  i2_specify=off  i2_priority=None  i2=0 A  i2_nominal_specify=off  i2_nominal_value=1  i2_nominal_unit=A  ife_specify=off  ife_priority=None  ife=0 A  ife_nominal_specify=off  ife_nominal_value=1  ife_nominal_unit=A  u1_specify=off  u1_priority=None  u1=0 V  u1_nominal_specify=off  u1_nominal_value=1  u1_nominal_unit=V  u2_specify=off  u2_priority=None  u2=0 V  u2_nominal_specify=off  u2_nominal_value=1  u2_nominal_unit=V
  ua : PMIOPort  Side=Right
  ub : PMIOPort  Port=2  Side=Right
  uc : PMIOPort  Port=3  Side=Right
  Ua : PMIOPort  Port=4  Side=Left
  Ub : PMIOPort  Port=5  Side=Left
  Uc : PMIOPort  Port=6  Side=Left
  connections:
  ph1/RConn1 -- ua/RConn1
  Electrical Reference1/LConn1 -- ph3/RConn2 -- ph2/RConn2 -- ph1/RConn2
  ph3/RConn1 -- uc/RConn1
  ph1/LConn1 -- Ua/RConn1 -- ph3/LConn2
  ph3/LConn1 -- Uc/RConn1 -- ph2/LConn2
  ph1/LConn2 -- Ub/RConn1 -- ph2/LConn1
  ph2/RConn1 -- ub/RConn1

== system power_system/grid/grid_emulator/3ph_Dyg/saturable_transformer_Dyn ==
  Electrical Reference1 : fl_lib/Electrical/Electrical Elements/Electrical Reference
  saturable_single_phase_transformer : saturable_single_phase_transformer/saturable_single_phase_transformer  enable_sat_m=param.grid.emu.trafo.enable_sat  m1=param.grid.emu.trafo.n1  m2=param.grid.emu.trafo.n2  rd1_trafo=param.grid.emu.trafo.Rd1  rd2_trafo=param.grid.emu.trafo.Rd2  ld1_trafo=param.grid.emu.trafo.Ld1  ld2_trafo=param.grid.emu.trafo.Ld2  rfe_trafo=param.grid.emu.trafo.Rfe1  area_core=param.grid.emu.trafo.core_area  length_core=param.grid.emu.trafo.core_length  mu0=param.grid.emu.trafo.mu0  mur_m=param.grid.emu.trafo.mur  phi_sat_m=param.grid.emu.trafo.psi*1.5
  saturable_single_phase_transformer1 : saturable_single_phase_transformer/saturable_single_phase_transformer  enable_sat_m=param.grid.emu.trafo.enable_sat  m1=param.grid.emu.trafo.n1  m2=param.grid.emu.trafo.n2  rd1_trafo=param.grid.emu.trafo.Rd1  rd2_trafo=param.grid.emu.trafo.Rd2  ld1_trafo=param.grid.emu.trafo.Ld1  ld2_trafo=param.grid.emu.trafo.Ld2  rfe_trafo=param.grid.emu.trafo.Rfe1  area_core=param.grid.emu.trafo.core_area  length_core=param.grid.emu.trafo.core_length  mu0=param.grid.emu.trafo.mu0  mur_m=param.grid.emu.trafo.mur  phi_sat_m=param.grid.emu.trafo.psi*1.5
  saturable_single_phase_transformer2 : saturable_single_phase_transformer/saturable_single_phase_transformer  enable_sat_m=param.grid.emu.trafo.enable_sat  m1=param.grid.emu.trafo.n1  m2=param.grid.emu.trafo.n2  rd1_trafo=param.grid.emu.trafo.Rd1  rd2_trafo=param.grid.emu.trafo.Rd2  ld1_trafo=param.grid.emu.trafo.Ld1  ld2_trafo=param.grid.emu.trafo.Ld2  rfe_trafo=param.grid.emu.trafo.Rfe1  area_core=param.grid.emu.trafo.core_area  length_core=param.grid.emu.trafo.core_length  mu0=param.grid.emu.trafo.mu0  mur_m=param.grid.emu.trafo.mur  phi_sat_m=param.grid.emu.trafo.psi*1.5
  ua : PMIOPort  Side=Right
  ub : PMIOPort  Port=2  Side=Right
  uc : PMIOPort  Port=3  Side=Right
  Ua : PMIOPort  Port=4  Side=Left
  Ub : PMIOPort  Port=5  Side=Left
  Uc : PMIOPort  Port=6  Side=Left
  connections:
  saturable_single_phase_transformer1/RConn1 -- ub/RConn1
  Ub/RConn1 -- saturable_single_phase_transformer1/LConn1 -- saturable_single_phase_transformer/LConn2
  Uc/RConn1 -- saturable_single_phase_transformer2/LConn1 -- saturable_single_phase_transformer1/LConn2
  Ua/RConn1 -- saturable_single_phase_transformer2/LConn2 -- saturable_single_phase_transformer/LConn1
  saturable_single_phase_transformer2/RConn1 -- uc/RConn1
  saturable_single_phase_transformer2/RConn2 -- Electrical Reference1/LConn1 -- saturable_single_phase_transformer1/RConn2 -- saturable_single_phase_transformer/RConn2
  saturable_single_phase_transformer/RConn1 -- ua/RConn1

== system power_system/grid/grid_emulator/3ph_Dyg/saturable_transformer_Dyn1 ==
  Dd : Subsystem
  Dyn : Subsystem
  ua : PMIOPort  Side=Right
  ub : PMIOPort  Port=2  Side=Right
  uc : PMIOPort  Port=3  Side=Right
  Ua : PMIOPort  Port=4  Side=Left
  Ub : PMIOPort  Port=5  Side=Left
  Uc : PMIOPort  Port=6  Side=Left
  connections:
  Dd/LConn1 -- Ua/RConn1
  Ub/RConn1 -- Dd/LConn2
  Uc/RConn1 -- Dd/LConn3
  ua/RConn1 -- Dyn/LConn1 -- Dd/RConn1
  Dd/RConn2 -- Dyn/LConn2 -- ub/RConn1
  uc/RConn1 -- Dyn/LConn3 -- Dd/RConn3

== system power_system/grid/grid_emulator/3ph_Dyg/saturable_transformer_Dyn1/Dd ==
  PS Terminator : fl_lib/Physical Signals/Sinks/PS Terminator
  PS Terminator1 : fl_lib/Physical Signals/Sinks/PS Terminator
  PS Terminator2 : fl_lib/Physical Signals/Sinks/PS Terminator
  T1 : three_phase_transformer_lib/Three-Phase Transformer Dd (delta primary, delta secondary)  Sr=param.grid.emu.trafo.pu.Sr A*V  V1=param.grid.emu.trafo.pu.V1 V  V2=param.grid.emu.trafo.pu.V2 V  fr=param.grid.emu.trafo.pu.fr Hz  clock_number=param.grid.emu.trafo.pu.clock  r1=param.grid.emu.trafo.pu.r1  l1=param.grid.emu.trafo.pu.l1  r2=param.grid.emu.trafo.pu.r2  l2=param.grid.emu.trafo.pu.l2  lm=param.grid.emu.trafo.pu.lm  lm0=param.grid.emu.trafo.pu.lm0  rfe=param.grid.emu.trafo.pu.rfe  iAB_specify=off  iAB_priority=None  iAB=0 A  iAB_nominal_specify=off  iAB_nominal_value=1  iAB_nominal_unit=A  iBC_specify=off  iBC_priority=None  iBC=0 A  iBC_nominal_specify=off  iBC_nominal_value=1  iBC_nominal_unit=A  iCA_specify=off  iCA_priority=None  iCA=0 A  iCA_nominal_specify=off  iCA_nominal_value=1  iCA_nominal_unit=A  i2ab_specify=off  i2ab_priority=None  i2ab=0 A  i2ab_nominal_specify=off  i2ab_nominal_value=1  i2ab_nominal_unit=A  i2bc_specify=off  i2bc_priority=None  i2bc=0 A  i2bc_nominal_specify=off  i2bc_nominal_value=1  i2bc_nominal_unit=A  i2ca_specify=off  i2ca_priority=None  i2ca=0 A  i2ca_nominal_specify=off  i2ca_nominal_value=1  i2ca_nominal_unit=A
  ua : PMIOPort  Side=Right
  Ua : PMIOPort  Port=2  Side=Left
  ub : PMIOPort  Port=3  Side=Right
  uc : PMIOPort  Port=4  Side=Right
  Ub : PMIOPort  Port=5  Side=Left
  Uc : PMIOPort  Port=6  Side=Left
  connections:
  T1/RConn3 -- uc/RConn1
  T1/RConn6 -- PS Terminator2/LConn1
  T1/LConn2 -- Ub/RConn1
  T1/RConn2 -- ub/RConn1
  PS Terminator/LConn1 -- T1/RConn4
  PS Terminator1/LConn1 -- T1/RConn5
  T1/LConn1 -- Ua/RConn1
  T1/RConn1 -- ua/RConn1
  T1/LConn3 -- Uc/RConn1
